simulink model "inverter"  (R2020a)
settings: Solver=VariableStepAuto  StartTime=0.0  StopTime=3  MaxStep=1e-7  RelTol=1e-7
undefined symbols (not defined in the file): Ion, Lithium
libraries: powerlib x9, simulink x2, electricdrivelib x1
settings Model: EnablePacing=on  PacingRate=10  Creator=siddyq  LastModifiedBy=siddyq

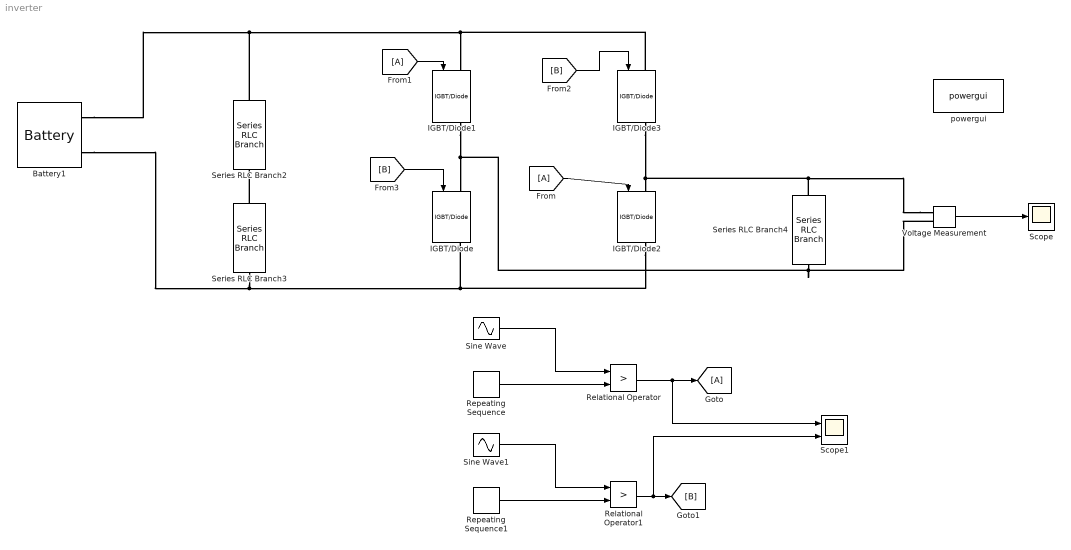
== system inverter ==
  Battery1 : electricdrivelib/Extra Sources/Battery  BatType=Lithium-Ion  ShowTempParam=off  ThermalPreset=no  ShowAgeParam=off  NomV=100  NomQ=100  SOC=100  Batt_Tr=1  PresetModel=on  MaxQ=100  MinV=75  FullV=116.3987  Dis_rate=43.4783  R=0.01  Normal_OP=90.4348  expZone="[108.0386      4.913043]"  current=[6.5 13 32.5]  Units=Time  Tci=20  NomT=20  T2=-30  MaxQ2=4.8  FullV2=7.1  Normal_OP2=5.655  expZone2="[6.58           1]"  Rca=0.6  ti=2000  Dp=0  Neq0=0  Tsim=1e6  Ta1=25  Qeol=5.4*0.9  Reol=0.013333*1.2  Char_age=[2.3478, 3]  Dis_age=[2.3478, 10]  N1=1500  N2=10500  N3=1000  N4=1400  Ta2=45  N5=950
  IGBT/Diode{,1..3} (4 alike) : powerlib/Power Electronics/IGBT//Diode  Ron=1e-3  Rs=1e5  Cs=inf  Measurements=on
  Relational Operator : RelationalOperator  Operator=>  OutDataTypeStr=boolean  RndMeth=Simplest
  Relational Operator1 : RelationalOperator  Operator=>  OutDataTypeStr=boolean  RndMeth=Simplest
  Repeating Sequence : simulink/Sources/Repeating Sequence  rep_seq_t=[0 0.02/40 0.02/20]  rep_seq_y=[0 1 0]
  Repeating Sequence1 : simulink/Sources/Repeating Sequence  rep_seq_t=[0 0.02/40 0.02/20]  rep_seq_y=[0 1 0]
  Scope : Scope
  Scope1 : Scope  NumInputPorts=2
  Series RLC Branch2 : powerlib/Elements/Series RLC Branch  LConnTagsString=__new0  RConnTagsString=__new0  BranchType=C  Resistance=1  Inductance=1e-3  SetiL0=off  InitialCurrent=0  Capacitance=1000e-6  Setx0=off  InitialVoltage=0  Measurements=None
  Series RLC Branch3 : powerlib/Elements/Series RLC Branch  LConnTagsString=__new0  RConnTagsString=__new0  BranchType=C  Resistance=1  Inductance=1e-3  SetiL0=off  InitialCurrent=0  Capacitance=1000e-6  Setx0=off  InitialVoltage=0  Measurements=None
  Series RLC Branch4 : powerlib/Elements/Series RLC Branch  LConnTagsString=__new0  RConnTagsString=__new0  BranchType=R  Resistance=10  Inductance=10e-3  SetiL0=off  InitialCurrent=0  Capacitance=1e-6  Setx0=off  InitialVoltage=0  Measurements=None
  Sine Wave : Sin  Frequency=100*pi  SampleTime=0
  Sine Wave1 : Sin  Frequency=100*pi  Phase=pi  SampleTime=0
  Voltage Measurement : powerlib/Measurements/Voltage Measurement  PhasorSimulation=off  OutputType=Complex  PSBequivalent=0
  powergui : powerlib/powergui  Priority=1  SimulationMode=Continuous  SampleTime=50e-6  frequency=60  Iterations=50  frequencyindice=0  Pbase=100e6  ErrMax=1e-4  UnitsV=kV  UnitsW=MW  buscounter=0  FunctionMessages=off  echomessages=off  EnableUseOfTLC=off  CurrentSourceSwitches=off  DisableSnubberDevices=off  DisableRonSwitches=off  DisableVfSwitches=off  DisplayEquations=off  AutomaticDiscreteSolvers=off  SolverType=Tustin/Backward Euler (TBE)  Interpol=off  ExternalGateDelay=off  methode=off  Ts=100  x0status=blocks  SPID=on  SwTol=0  HookPort=off  NonlinearTolerance=1e-4  nMaxIteration=100  ContinueOnMaxIteration=off  RestoreLinks=warning  ResistiveCurrentMeasurement=off  Frange=[0:2:500]  Ylog=off  Xlog=on  ShowGrid=off  save=off  variable=ZData  structure=0  ZoomFFT=off  StartTime=0.0  cycles=1  DisplayStyle=1  fundamental=60  FreqAxis=off  MaxFrequency=1000  frequencyindicesteady=1  RmsSteady=1  display=off
  wires:
  Voltage Measurement/1 -> Scope/1
  [B] -> IGBT/Diode3/1
  [A] -> IGBT/Diode2/1
  Sine Wave/1 -> Relational Operator/1
  Repeating Sequence/1 -> Relational Operator/2
  [A] -> IGBT/Diode1/1
  Repeating Sequence1/1 -> Relational Operator1/2
  Relational Operator1/1 -> Scope1/2, [B]
  [B] -> IGBT/Diode/1
  Relational Operator/1 -> Scope1/1, [A]
  Sine Wave1/1 -> Relational Operator1/1
  connections:
  Voltage Measurement/LConn1 -- IGBT/Diode3/RConn1 -- IGBT/Diode2/LConn1 -- Series RLC Branch4/RConn1
  Battery1/LConn1 -- Series RLC Branch2/LConn1 -- IGBT/Diode3/LConn1 -- IGBT/Diode1/LConn1
  Battery1/LConn2 -- Series RLC Branch3/RConn1 -- IGBT/Diode2/RConn1 -- IGBT/Diode/RConn1
  Series RLC Branch3/LConn1 -- Series RLC Branch2/RConn1
  IGBT/Diode1/RConn1 -- Voltage Measurement/LConn2 -- Series RLC Branch4/LConn1 -- IGBT/Diode/LConn1
